simulink model "Single_Phase_Induction_Motor_DPWM"  (R2023b)
settings: Solver=VariableStepAuto  StartTime=0.0  StopTime=0.5  RelTol=1e-3
libraries: spsMeanLib x2, spsRMSLib x2, spsVoltageMeasurementLib x2, spsCurrentMeasurementLib x2, spsControlledVoltageSourceLib x2, spsSeriesRLCBranchLib x2, spsDCVoltageSourceLib x1, spsUniversalBridgeLib x1, spspowerguiLib x1, simulink x1, eeTransforms x1, slpidlib x1
settings Model: SimulationMode=accelerator  Creator=Qu  LastModifiedBy=Qu
settings SolverCC: ZeroCrossAlgorithm=Adaptive
settings DebuggingCC: IgnoredZcDiagnostic=none

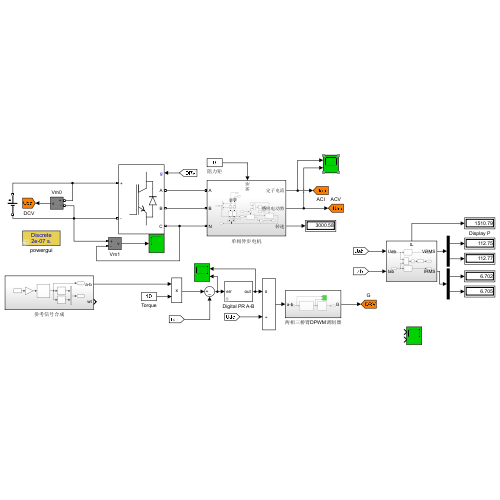
[thumbnail: Simulink's stored preview of the top-level diagram]
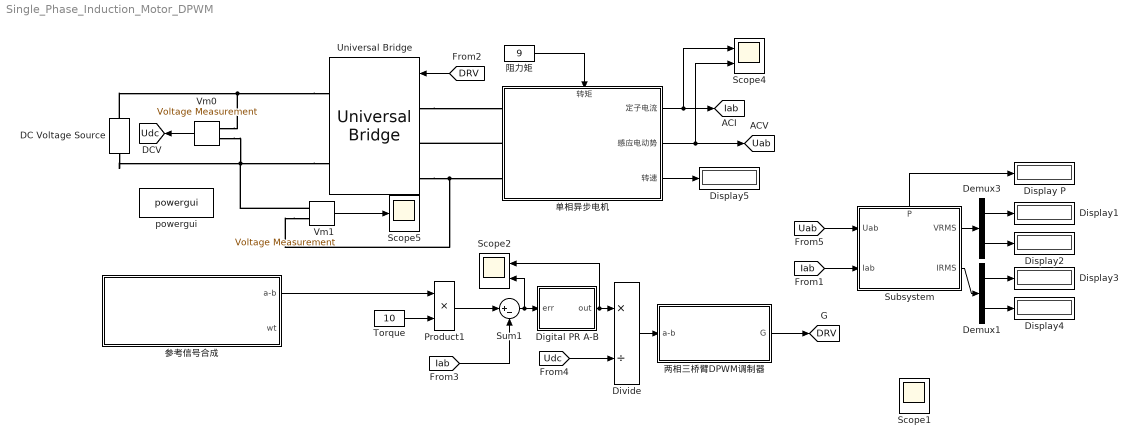
== system Single_Phase_Induction_Motor_DPWM ==
  DC Voltage Source : spsDCVoltageSourceLib/DC Voltage Source  Amplitude=400  Measurements=None
  Demux1 : Demux  Outputs=2
  Demux3 : Demux  Outputs=2
  Digital PR A-B : Subsystem  mask{Kp=6, Kr=400, Wc=5, Ts=1/20000, Upper=500, Lower=-500}
      mask DialogControl ParameterGroupVar Prompt: 参数
  Display P : Display
      settings: Format=bank
  Display{1..5} (5 alike) : Display
      Display1 settings: Format=bank
      Display2 settings: Format=bank
      Display5 settings: Format=bank
  Divide : Product  Inputs=*/
  Product1 : Product
  Scope1 : Scope  NumInputPorts=2
  Scope2 : Scope  NumInputPorts=2
  Scope4 : Scope  NumInputPorts=2
  Scope5 : Scope
  Subsystem : Subsystem
      settings: PortSchema="{\"entries\":[{\"content\":{\"sides\":[{\"content\":{\"connectorIds\":[\"In1\",\"In2\"]},\"type\":\"ConnectorPlacement.EquallySpacedRectSide\",\"uuid\":\"1a30de24-3f6a-4a71-ab9e-a89e986dc660\"},{\"content\":{\"connectorIds\":[\"Out1\",\"Out2\"],\"side\":\"RIGHT\"},\"type\":\"ConnectorPlacement.EquallySpacedRectSide\",\"uuid\":\"54b35498-05dd-4d62-910a-7356b29a6052\"},{\"content\":{\"connectorIds\":[\"Out3\"],\"side\":\"TOP\"},\"type\":\"ConnectorPlacement.EquallySpacedRectSide\",\"uuid\":\"d7674575-867d-4c16-b3d3-3c0c8548789c\"}]},\"type\":\"ConnectorPlacement.EquallySpacedConnector\",\"uuid\":\"2766d3bc-f88a-4d97-ac9a-989f58a0c4f0\"}],\"packageUris\":[\"http://schema.mathworks.com/mf0/Connector/R2020b\"],\"version\":\"1.0\"}"
  Sum1 : Sum  Inputs=|+-
  Torque : Constant  Value=10
  Universal Bridge : spsUniversalBridgeLib/Universal Bridge  Arms=3  SnubberResistance=1e5  SnubberCapacitance=inf  Device=IGBT / Diodes  Ron=1e-3  Lon=0  ForwardVoltages="[  1  1  ]"  ForwardVoltage=0  GTOparameters=[ 10e-6 , 20e-6 ]  IGBTparameters=[ 1e-6 , 2e-6 ]  Measurements=None  Measurements_2=None  converterType=Rectifier
  Vm0 : spsVoltageMeasurementLib/Voltage Measurement  PhasorSimulation=off  OutputType=Complex  PSBequivalent=0
  Vm1 : spsVoltageMeasurementLib/Voltage Measurement  PhasorSimulation=off  OutputType=Complex  PSBequivalent=0
  powergui : spspowerguiLib/powergui  SimulationMode=Discrete  SampleTime=2e-7  frequency=60  Iterations=50  frequencyindice=0  Pbase=100e6  ErrMax=1e-4  UnitsV=kV  UnitsW=MW  buscounter=0  FunctionMessages=off  echomessages=off  EnableUseOfTLC=off  CurrentSourceSwitches=off  DisableSnubberDevices=off  DisableRonSwitches=off  DisableVfSwitches=off  DisplayEquations=off  AutomaticDiscreteSolvers=off  SolverType=Tustin/Backward Euler (TBE)  Interpol=off  ExternalGateDelay=off  methode=off  Ts=0  x0status=blocks  SPID=off  SwTol=0  HookPort=off  NonlinearTolerance=1e-4  nMaxIteration=100  ContinueOnMaxIteration=off  RestoreLinks=warning  ResistiveCurrentMeasurement=off  Frange=[0:2:500]  Ylog=off  Xlog=on  ShowGrid=off  save=off  variable=ZData  structure=QQQQQ  ZoomFFT=off  StartTime=0.5  cycles=15  DisplayStyle=1  fundamental=50  FreqAxis=off  MaxFrequency=1000  frequencyindicesteady=1  RmsSteady=1  display=off
  两相三桥臂DPWM调制器 : Subsystem
  单相异步电机 : Subsystem
      settings: PortSchema="{\"entries\":[{\"content\":{\"sides\":[{\"content\":{\"connectorIds\":[\"LConn1\",\"LConn2\",\"LConn3\"]},\"type\":\"ConnectorPlacement.EquallySpacedRectSide\",\"uuid\":\"8c540c10-daf6-43f0-a361-fb5761fea74a\"},{\"content\":{\"connectorIds\":[\"Out1\",\"Out2\",\"Out3\"],\"side\":\"RIGHT\"},\"type\":\"ConnectorPlacement.EquallySpacedRectSide\",\"uuid\":\"ed6e8eeb-f359-49e0-9e7e-9ec6a0e9de26\"},{\"content\":{\"connectorIds\":[\"In1\"],\"side\":\"TOP\"},\"type\":\"ConnectorPlacement.EquallySpacedRectSide\",\"uuid\":\"75c389a8-3525-4841-a458-838b002b3a73\"}]},\"type\":\"ConnectorPlacement.EquallySpacedConnector\",\"uuid\":\"bcd27d16-37c3-48dd-9d92-cb99fef489c7\"}],\"packageUris\":[\"http://schema.mathworks.com/mf0/Connector/R2020b\"],\"version\":\"1.0\"}"
  参考信号合成 : Subsystem
  阻力矩 : Constant  Value=9
  tag scope: DRV=global, Iab=global, Uab=global, Udc=global
  wires:
  Torque/1 -> Product1/2
  单相异步电机/1(定子电流) -> [Iab], Scope4/1
  单相异步电机/2(感应电动势) -> [Uab], Scope4/2
  Vm0/1 -> [Udc]
  Sum1/1 -> Scope2/2, Digital PR A-B/1(err)
  Demux3/1 -> Display1/1
  Subsystem/3(P) -> Display P/1
  Demux1/2 -> Display4/1
  Subsystem/2(IRMS) -> Demux1/1
  Subsystem/1(VRMS) -> Demux3/1
  Demux3/2 -> Display2/1
  [DRV] -> Universal Bridge/1
  [Uab] -> Subsystem/1(Uab)
  [Udc] -> Divide/2
  两相三桥臂DPWM调制器/1(G) -> [DRV]
  Vm1/1 -> Scope5/1
  [Iab] -> Subsystem/2(Iab)
  Digital PR A-B/1(out) -> Scope2/1, Divide/1
  [Iab] -> Sum1/2
  Demux1/1 -> Display3/1
  单相异步电机/3(转速) -> Display5/1
  阻力矩/1 -> 单相异步电机/1(转矩)
  参考信号合成/1(a-b) -> Product1/1
  Divide/1 -> 两相三桥臂DPWM调制器/1(a-b)
  Product1/1 -> Sum1/1
  connections:
  Vm1/LConn2 -- Universal Bridge/LConn3 -- 单相异步电机/LConn3
  Universal Bridge/RConn1 -- Vm0/LConn1 -- DC Voltage Source/RConn1
  Universal Bridge/RConn2 -- DC Voltage Source/LConn1 -- Vm0/LConn2 -- Vm1/LConn1
  Universal Bridge/LConn1 -- 单相异步电机/LConn1
  单相异步电机/LConn2 -- Universal Bridge/LConn2

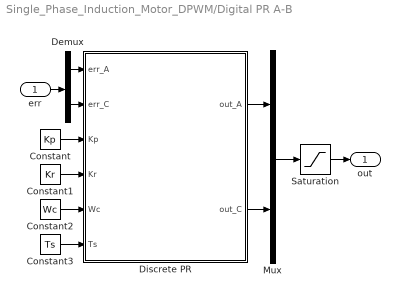
== system Single_Phase_Induction_Motor_DPWM/Digital PR A-B ==
  err : Inport
  Constant : Constant  Value=Kp
  Constant1 : Constant  Value=Kr
  Constant2 : Constant  Value=Wc
  Constant3 : Constant  Value=Ts
  Demux : Demux  Outputs=2
  Discrete PR : MATLAB Function  TreatAsAtomicUnit=on
  Mux : Mux  Inputs=2
  Saturation : Saturate  UpperLimit=Upper  LowerLimit=Lower
  out : Outport
  wires:
  Constant1/1 -> Discrete PR/4(Kr)
  Constant3/1 -> Discrete PR/6(Ts)
  Constant/1 -> Discrete PR/3(Kp)
  Constant2/1 -> Discrete PR/5(Wc)
  Demux/1 -> Discrete PR/1(err_A)
  err/1 -> Demux/1
  Demux/2 -> Discrete PR/2(err_C)
  Discrete PR/1(out_A) -> Mux/1
  Discrete PR/2(out_C) -> Mux/2
  Mux/1 -> Saturation/1
  Saturation/1 -> out/1

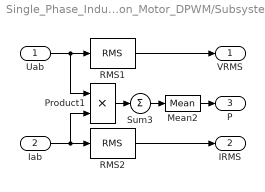
== system Single_Phase_Induction_Motor_DPWM/Subsystem ==
  Uab : Inport
  Iab : Inport  Port=2
  Mean2 : spsMeanLib/Mean  Freq=50  Vinit=0  Ts=0
  Product1 : Product
  RMS1 : spsRMSLib/RMS  TrueRMS=on  Freq=50  RMSInit=0  Ts=0
  RMS2 : spsRMSLib/RMS  TrueRMS=on  Freq=50  RMSInit=0  Ts=0
  Sum3 : Sum  Inputs=+
  VRMS : Outport
  IRMS : Outport  Port=2
  P : Outport  Port=3
  wires:
  Uab/1 -> Product1/1, RMS1/1
  RMS2/1 -> IRMS/1
  Sum3/1 -> Mean2/1
  Mean2/1 -> P/1
  Iab/1 -> RMS2/1, Product1/2
  Product1/1 -> Sum3/1
  RMS1/1 -> VRMS/1

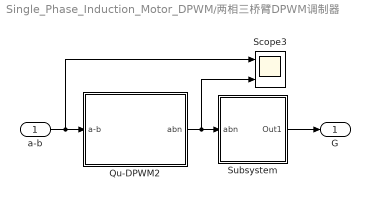
== system Single_Phase_Induction_Motor_DPWM/两相三桥臂DPWM调制器 ==
  a-b : Inport
  Qu-DPWM2 : Subsystem
  Scope3 : Scope  NumInputPorts=2
  Subsystem : Subsystem
  G : Outport
  wires:
  Subsystem/1(Out1) -> G/1
  a-b/1 -> Scope3/1, Qu-DPWM2/1(a-b)
  Qu-DPWM2/1(abn) -> Scope3/2, Subsystem/1(abn)

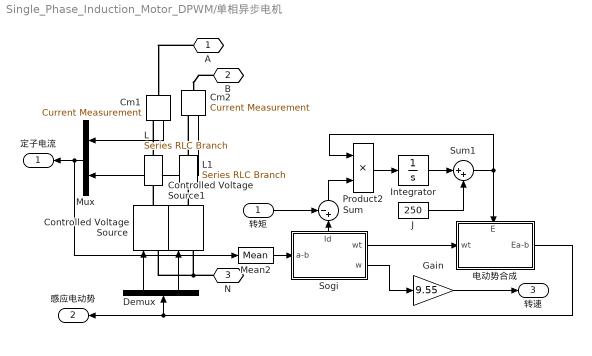
== system Single_Phase_Induction_Motor_DPWM/单相异步电机 ==
  转矩 : Inport
  Cm1 : spsCurrentMeasurementLib/Current Measurement  PhasorSimulation=off  OutputType=Complex  PSBequivalent=0
  Cm2 : spsCurrentMeasurementLib/Current Measurement  PhasorSimulation=off  OutputType=Complex  PSBequivalent=0
  Controlled Voltage Source : spsControlledVoltageSourceLib/Controlled Voltage Source  Initialize=on  Source_Type=AC  Amplitude=0  Phase=0  Frequency=0  Measurements=None
  Controlled Voltage Source1 : spsControlledVoltageSourceLib/Controlled Voltage Source  Initialize=on  Source_Type=AC  Amplitude=0  Phase=0  Frequency=0  Measurements=None
  Demux : Demux  Outputs=2
  Gain : Gain  Gain=9.55
  Integrator : Integrator
  J : Constant  Value=250
  L : spsSeriesRLCBranchLib/Series RLC Branch  LConnTagsString=__new0  RConnTagsString=__new0  BranchType=RL  Resistance=1  Inductance=0.005  SetiL0=off  InitialCurrent=0  Capacitance=33e-9  Setx0=off  InitialVoltage=0  Measurements=None
  L1 : spsSeriesRLCBranchLib/Series RLC Branch  LConnTagsString=__new0  RConnTagsString=__new0  BranchType=RL  Resistance=1  Inductance=0.005  SetiL0=off  InitialCurrent=0  Capacitance=33e-9  Setx0=off  InitialVoltage=0  Measurements=None
  Mean2 : spsMeanLib/Mean  Freq=10000  Vinit=1  Ts=0
  Mux : Mux  Inputs=2
  Product2 : Product
  Sogi : Subsystem
      settings: PortSchema="{\"entries\":[{\"content\":{\"sides\":[{\"content\":{\"connectorIds\":[\"In1\"]},\"type\":\"ConnectorPlacement.EquallySpacedRectSide\",\"uuid\":\"a13447a4-6888-491d-ad9a-e2350e48b0f3\"},{\"content\":{\"connectorIds\":[\"Out1\",\"Out2\"],\"side\":\"RIGHT\"},\"type\":\"ConnectorPlacement.EquallySpacedRectSide\",\"uuid\":\"ae3031e5-97cb-48de-99c1-36b9e64fdead\"},{\"content\":{\"connectorIds\":[\"Out3\"],\"side\":\"TOP\"},\"type\":\"ConnectorPlacement.EquallySpacedRectSide\",\"uuid\":\"441320d0-6b7a-45af-b050-5b8e815e10d8\"},{\"content\":{\"side\":\"BOTTOM\"},\"type\":\"ConnectorPlacement.EquallySpacedRectSide\",\"uuid\":\"0bec7bb7-dec1-400f-b0db-7d20f1493311\"}]},\"type\":\"ConnectorPlacement.EquallySpacedConnector\",\"uuid\":\"58db6bd9-1292-4ed1-a818-e1ef6e1eca54\"}],\"packageUris\":[\"http://schema.mathworks.com/mf0/Connector/R2020b\"],\"version\":\"1.0\"}"
  Sum : Sum  Inputs=-+|
  Sum1 : Sum  Inputs=|++
  电动势合成 : Subsystem
      settings: PortSchema="{\"entries\":[{\"content\":{\"sides\":[{\"content\":{\"connectorIds\":[\"In1\"]},\"type\":\"ConnectorPlacement.EquallySpacedRectSide\",\"uuid\":\"a13447a4-6888-491d-ad9a-e2350e48b0f3\"},{\"content\":{\"connectorIds\":[\"Out1\"],\"side\":\"RIGHT\"},\"type\":\"ConnectorPlacement.EquallySpacedRectSide\",\"uuid\":\"ae3031e5-97cb-48de-99c1-36b9e64fdead\"},{\"content\":{\"connectorIds\":[\"In2\"],\"side\":\"TOP\"},\"type\":\"ConnectorPlacement.EquallySpacedRectSide\",\"uuid\":\"441320d0-6b7a-45af-b050-5b8e815e10d8\"}]},\"type\":\"ConnectorPlacement.EquallySpacedConnector\",\"uuid\":\"58db6bd9-1292-4ed1-a818-e1ef6e1eca54\"}],\"packageUris\":[\"http://schema.mathworks.com/mf0/Connector/R2020b\"],\"version\":\"1.0\"}"
  A : PMIOPort  Side=Left
  B : PMIOPort  Port=2  Side=Left
  N : PMIOPort  Port=3  Side=Left
  定子电流 : Outport
  感应电动势 : Outport  Port=2
  转速 : Outport  Port=3
  wires:
  Demux/1 -> Controlled Voltage Source/1
  Demux/2 -> Controlled Voltage Source1/1
  Cm1/1 -> Mux/1
  Cm2/1 -> Mux/2
  Mux/1 -> 定子电流/1, Mean2/1
  Mean2/1 -> Sogi/1(a-b)
  电动势合成/1(Ea-b) -> Demux/1, 感应电动势/1
  Product2/1 -> Integrator/1
  Integrator/1 -> Sum1/1
  J/1 -> Sum1/2
  Sum1/1 -> 电动势合成/2(E), Product2/1
  Sogi/1(wt) -> 电动势合成/1(wt)
  Sogi/3(Id) -> Sum/2
  Sum/1 -> Product2/2
  转矩/1 -> Sum/1
  Gain/1 -> 转速/1
  Sogi/2(w) -> Gain/1
  connections:
  N/RConn1 -- Controlled Voltage Source1/LConn1 -- Controlled Voltage Source/LConn1
  A/RConn1 -- Cm1/LConn1
  Controlled Voltage Source/RConn1 -- L/RConn1
  L/LConn1 -- Cm1/RConn1
  L1/LConn1 -- Cm2/RConn1
  Controlled Voltage Source1/RConn1 -- L1/RConn1
  B/RConn1 -- Cm2/LConn1

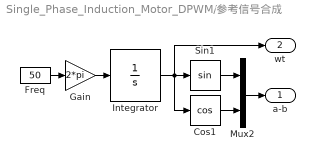
== system Single_Phase_Induction_Motor_DPWM/参考信号合成 ==
  Cos1 : Trigonometry  Operator=cos
  Freq : Constant  Value=50
  Gain : Gain  Gain=2*pi
  Integrator : Integrator  UpperSaturationLimit=65536  LowerSaturationLimit=0  WrapState=on  WrappedStateUpperValue=2*pi  WrappedStateLowerValue=0
  Mux2 : Mux  Inputs=2
  Sin1 : Trigonometry
  a-b : Outport
  wt : Outport  Port=2
  wires:
  Gain/1 -> Integrator/1
  Freq/1 -> Gain/1
  Integrator/1 -> Cos1/1, wt/1, Sin1/1
  Sin1/1 -> Mux2/1
  Cos1/1 -> Mux2/2
  Mux2/1 -> a-b/1

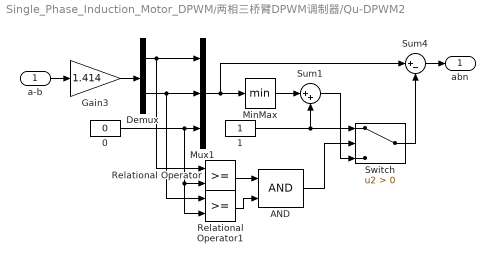
== system Single_Phase_Induction_Motor_DPWM/两相三桥臂DPWM调制器/Qu-DPWM2 ==
  a-b : Inport
  0 : Constant  Value=0
  1 : Constant
  AND : Logic  IconShape=distinctive  AllPortsSameDT=off  OutDataTypeStr=boolean
  Demux : Demux  Outputs=2
  Gain3 : Gain  Gain=1.414
  MinMax : MinMax
  Mux1 : Mux  Inputs=3
  Relational Operator : RelationalOperator  OutDataTypeStr=boolean  InputSameDT=off
  Relational Operator1 : RelationalOperator  OutDataTypeStr=boolean  InputSameDT=off
  Sum1 : Sum  Inputs=|++
  Sum4 : Sum  Inputs=|+-
  Switch : Switch  Criteria=u2 > Threshold  SaturateOnIntegerOverflow=off  InputSameDT=off
  abn : Outport
  wires:
  a-b/1 -> Gain3/1
  Mux1/1 -> Sum4/1, MinMax/1
  Demux/1 -> Relational Operator/1, Mux1/1
  Demux/2 -> Relational Operator1/1, Mux1/2
  0/1 -> Relational Operator1/2, Relational Operator/2, Mux1/3
  Gain3/1 -> Demux/1
  Relational Operator/1 -> AND/1
  Relational Operator1/1 -> AND/2
  MinMax/1 -> Sum1/1
  1/1 -> Switch/1, Sum1/2
  AND/1 -> Switch/2
  Switch/1 -> Sum4/2
  Sum4/1 -> abn/1
  Sum1/1 -> Switch/3

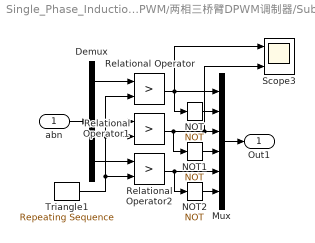
== system Single_Phase_Induction_Motor_DPWM/两相三桥臂DPWM调制器/Subsystem ==
  abn : Inport
  Demux : Demux  Outputs=3
  Mux : Mux  Inputs=6
  NOT : Logic  Operator=NOT  IconShape=distinctive  AllPortsSameDT=off  OutDataTypeStr=boolean
  NOT1 : Logic  Operator=NOT  IconShape=distinctive  AllPortsSameDT=off  OutDataTypeStr=boolean
  NOT2 : Logic  Operator=NOT  IconShape=distinctive  AllPortsSameDT=off  OutDataTypeStr=boolean
  Relational Operator : RelationalOperator  Operator=>  OutDataTypeStr=boolean  InputSameDT=off
  Relational Operator1 : RelationalOperator  Operator=>  OutDataTypeStr=boolean  InputSameDT=off
  Relational Operator2 : RelationalOperator  Operator=>  OutDataTypeStr=boolean  InputSameDT=off
  Scope3 : Scope  NumInputPorts=2
  Triangle1 : simulink/Sources/Repeating Sequence  rep_seq_t=[0 1/20000/2 1/20000]  rep_seq_y=[-1 1 -1]
  Out1 : Outport
  wires:
  NOT/1 -> Mux/2
  Relational Operator2/1 -> NOT2/1, Mux/5
  Triangle1/1 -> Relational Operator/2, Relational Operator1/2, Relational Operator2/2
  NOT2/1 -> Mux/6
  Relational Operator1/1 -> NOT1/1, Scope3/2, Mux/3
  Demux/3 -> Relational Operator2/1
  NOT1/1 -> Mux/4
  Mux/1 -> Out1/1
  Demux/2 -> Relational Operator1/1
  abn/1 -> Demux/1
  Demux/1 -> Relational Operator/1
  Relational Operator/1 -> NOT/1, Scope3/1, Mux/1

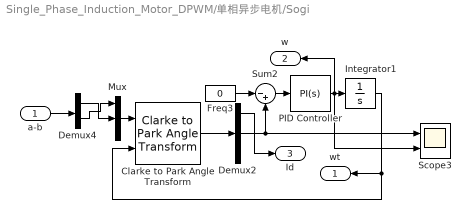
== system Single_Phase_Induction_Motor_DPWM/单相异步电机/Sogi ==
  a-b : Inport
  Clarke to Park Angle Transform : eeTransforms/Clarke to Park Angle Transform  AxisAlignment=D-axis
      settings: LibrarySourceBlock=|
      | ee_sl_lib/Mathematical
      | Transforms/Clarke to Park
      | Angle Transform
  Demux2 : Demux  Outputs=3
  Demux4 : Demux  Outputs=2
  Freq3 : Constant  Value=0
  Integrator1 : Integrator  UpperSaturationLimit=2*pi  LowerSaturationLimit=0  WrapState=on  WrappedStateUpperValue=2*pi  WrappedStateLowerValue=0
  Mux : Mux  Inputs=3
  PID Controller : slpidlib/PID Controller  Controller=PI  Form=Parallel  TimeDomain=Continuous-time  UseExternalTs=off  SampleTime=-1  IntegratorMethod=Forward Euler  FilterMethod=Forward Euler  ControllerParametersSource=internal  P=1  I=10  UseKiTs=off  D=0  N=100  UseFilter=on  TunerSelectOption=Transfer Function Based (PID Tuner App)  InitialConditionSource=internal  InitialConditionForIntegrator=314  InitialConditionForFilter=0  DifferentiatorICPrevScaledInput=0  ExternalReset=none  TrackingMode=off  Kt=1  LimitOutput=off  SatLimitsSource=internal  UpperSaturationLimit=inf  LowerSaturationLimit=-inf  LinearizeAsGain=on  AntiWindupMode=none  Kb=1  LimitIntegrator=off  UpperIntegratorSaturationLimit=inf  LowerIntegratorSaturationLimit=-inf  POutMin=[]  POutMax=[]  IOutMin=[]  IOutMax=[]  DOutMin=[]  DOutMax=[]  NOutMin=[]  NOutMax=[]  SumOutMin=[]  SumOutMax=[]  SaturationOutMin=[]  SaturationOutMax=[]  PParamMin=[]  PParamMax=[]  IParamMin=[]  IParamMax=[]  DParamMin=[]  DParamMax=[]  NParamMin=[]  NParamMax=[]  KbParamMin=[]  KbParamMax=[]  KtParamMin=[]  KtParamMax=[]  KbOutMin=[]  KbOutMax=[]  KtOutMin=[]  KtOutMax=[]  IntegratorOutMin=[]  IntegratorOutMax=[]  FilterOutMin=[]  FilterOutMax=[]  SumI1OutMin=[]  SumI1OutMax=[]  SumI2OutMin=[]  SumI2OutMax=[]  SumI3OutMin=[]  SumI3OutMax=[]  SumI4OutMin=[]  SumI4OutMax=[]  SumDOutMin=[]  SumDOutMax=[]  DifferentiatorOutMin=[]  DifferentiatorOutMax=[]  FilterDiffOutCoefMin=[]  FilterDiffOutCoefMax=[]  ReciprocalOutMin=[]  ReciprocalOutMax=[]  SumDenOutMin=[]  SumDenOutMax=[]  SumNumOutMin=[]  SumNumOutMax=[]  DivideOutMin=[]  DivideOutMax=[]  UdiffTsProdOutMin=[]  UdiffTsProdOutMax=[]  NTsProdOutMin=[]  NTsProdOutMax=[]  UintegralTsProdOutMin=[]  UintegralTsProdOutMax=[]  UngainTsProdOutMin=[]  UngainTsProdOutMax=[]  ClampingZeroOutDataTypeStr=Inherit: Inherit via back propagation  ClampingZeroOutMin=[]  ClampingZeroOutMax=[]  FilterDenConstantOutDataTypeStr=Inherit: Inherit via back propagation  FilterDenConstantOutMin=[]  FilterDenConstantOutMax=[]  PCopyOutDataTypeStr=Inherit: Inherit via back propagation  PCopyOutMin=[]  PCopyOutMax=[]  NCopyOutDataTypeStr=Inherit: Inherit via back propagation  NCopyOutMin=[]  NCopyOutMax=[]  IntegratorContinuousStateAttributes=''  IntegratorStateMustResolveToSignalObject=off  IntegratorRTWStateStorageClass=Auto  FilterContinuousStateAttributes=''  FilterStateMustResolveToSignalObject=off  FilterRTWStateStorageClass=Auto  ParallelPVariant=InternalParameters  IdealPVariant=Disabled  IVariant=InternalParameters  DVariant=Disabled  IntegratorVariant=Continuous  SatVariant=Disabled  AWVariant=Passthrough  PCopyVariant=Disabled  TRVariant=Disabled  FdbkBlocksVariant=Forward  IdealPFdbkVariant=Disabled  SatFdbkVariant=Disabled  DerivativeFilterVariant=Disabled  NVariant=Disabled  NCopyVariant=Disabled_SignalSpec  FilterICVariant=Disabled  IntegratorICVariant=InternalICs  ExternalResetVariant=Disabled  TRSumVariant=Passthrough  SumFdbkVariant=Disabled  SumVariant=Sum_PI  TsampFilterVariant=InternalTs  TsampNgainVariant=Passthrough  TsampIntegralVariant=Disabled_SignalSpec  ExternalSaturationOutDataTypeStr=Inherit: Same as second input
  Scope3 : Scope  NumInputPorts=2
  Sum2 : Sum  Inputs=|-+
  wt : Outport
  w : Outport  Port=2
  Id : Outport  Port=3
  wires:
  Clarke to Park Angle Transform/1 -> Demux2/1
  Mux/1 -> Clarke to Park Angle Transform/1
  Freq3/1 -> Sum2/1
  Demux2/2 -> Scope3/1, Sum2/2
  Demux4/1 -> Mux/2
  PID Controller/1 -> Scope3/2, w/1, Integrator1/1
  Demux4/2 -> Mux/1
  Sum2/1 -> PID Controller/1
  a-b/1 -> Demux4/1
  Integrator1/1 -> Clarke to Park Angle Transform/2, wt/1
  Demux2/1 -> Id/1

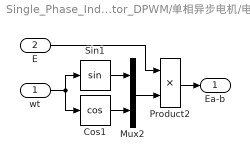
== system Single_Phase_Induction_Motor_DPWM/单相异步电机/电动势合成 ==
  wt : Inport
  E : Inport  Port=2
  Cos1 : Trigonometry  Operator=cos
  Mux2 : Mux  Inputs=2
  Product2 : Product
  Sin1 : Trigonometry
  Ea-b : Outport
  wires:
  wt/1 -> Cos1/1, Sin1/1
  Sin1/1 -> Mux2/1
  Cos1/1 -> Mux2/2
  Mux2/1 -> Product2/2
  E/1 -> Product2/1
  Product2/1 -> Ea-b/1

== matlab function Single_Phase_Induction_Motor_DPWM/Digital PR A-B/Discrete PR ==
  settings: updateMethod=DISCRETE  sampleTime=Ts
  data: err_A input; err_C input; out_A output; Kp input; Kr input; Wc input; Ts input; out_C output
function [out_A, out_C] = fcn(err_A, err_C, Kp, Kr, Wc, Ts)

W0 = 50*2*pi;

%%定义三相静态变量
persistent err_A1;
persistent err_A2;
persistent out_A1;
persistent out_A2;

persistent err_C1;
persistent err_C2;
persistent out_C1;
persistent out_C2;

%%对三相静态变量初始化
if isempty(err_A1)
    err_A1 = 0;
end
if isempty(err_A2)
    err_A2 = 0;
end
if isempty(out_A1)
    out_A1 = 0;
end
if isempty(out_A2)
    out_A2 = 0;
end


if isempty(err_C1)
    err_C1 = 0;
end
if isempty(err_C2)
    err_C2 = 0;
end
if isempty(out_C1)
    out_C1 = 0;
end
if isempty(out_C2)
    out_C2 = 0;
end

%%Discrete
t1 = Wc * Ts;
t2 = W0^2 * Ts^2;
t3 = t2 + 4*t1 + 4;

b0 = (Kp*t2 + 4*(Kp+Kr)*t1 + 4*Kp) / t3;
b1 = (2*Kp*t2 - 8*Kp) / t3;
b2 = (Kp*t2 + 4*Kp - 4*(Kp+Kr)*t1) / t3;
a1 = (2*t2 - 8) / t3;
a2 = (t2 - 4*t1 + 4) / t3;

%%计算三相输出量
out_A = b0*err_A + b1*err_A1 + b2*err_A2 - a1*out_A1 - a2*out_A2;
out_A2 = out_A1;
out_A1 = out_A;
err_A2 = err_A1;
err_A1 = err_A;


out_C = b0*err_C + b1*err_C1 + b2*err_C2 - a1*out_C1 - a2*out_C2;
out_C2 = out_C1;
out_C1 = out_C;
err_C2 = err_C1;
err_C1 = err_C;
